simulink model "AvonGasTurbineFAult"  (R2016b)
settings: Solver=ode45  StartTime=0.0  StopTime=3000  FixedStep=1  RelTol=1e-3  EnableMultiTasking=on
InitFcn:
  | warning off
undefined symbols (not defined in the file or in its folder): flagFalut, thresholdbound, xflt
libraries: neural x74, fuzblock x6, simulink x5
(part 3 of 4)

== system AvonGasTurbineFAult/FG_valve/Layer 2/LW{2,1} ==
  "ad{2,1}" : Inport  PortDimensions=10
      mask Display: e = 0.06;c1 = [120 230 180]/255;c2 = ([120 230 180]+0)/(256+128);c3 = ([120 230 180]+128)/(256+128);patch([0 1 1 0],[0 0 1 1],c1);patch([0 1 1 1-e 1-e 0+e],[0 0 1 1-e 0+e 0+e],c2);patch([0 0 1 1-e 0+e 0+e],[0 1 1 1-e 1-e 0+e],c3);plot([0 1 1 0 0],[0 0 1 1 0]);
  "IW{2,1}(1,:)'" : Constant  Value=[-3.0687263870923882;-0.58010050017961035;-1.6732268530537433;1.1111209811250431;-3.7658607876141885;4.9608535154988296;-4.0233887362216931;0.877154954427946;-0.007111666457348894;-2.3567838960567342]
      mask Display: e = 0.06;c1 = [120 150 230]/255;c2 = ([120 150 230]+0)/383;c3 = ([120 150 230]+128)/383;patch([0 1 1 0],[0 0 1 1],c1);patch([0 1 1 1-e 1-e 0+e],[0 0 1 1-e 0+e 0+e],c2);patch([0 0 1 1-e 0+e 0+e],[0 1 1 1-e 1-e 0+e],c3);plot([0 1 1 0 0],[0 0 1 1 0]);disp('weights');
  "IW{2,1}(2,:)'" : Constant  Value=[2.944755261970526;0.25323877938735545;-0.37016123547701313;-0.49590463373628868;-1.4090557527728114;0.65410480645354996;-1.1498049344641088;1.9422996654200746;1.3204846277569529;-1.2106760170631452]
      mask Display: e = 0.06;c1 = [120 150 230]/255;c2 = ([120 150 230]+0)/383;c3 = ([120 150 230]+128)/383;patch([0 1 1 0],[0 0 1 1],c1);patch([0 1 1 1-e 1-e 0+e],[0 0 1 1-e 0+e 0+e],c2);patch([0 0 1 1-e 0+e 0+e],[0 1 1 1-e 1-e 0+e],c3);plot([0 1 1 0 0],[0 0 1 1 0]);disp('weights');
  "IW{2,1}(3,:)'" : Constant  Value=[-0.90291968530259159;1.9861760248636133;-0.86703740713984767;-1.2961573454155009;4.5697519100862136;-0.36889440045356731;2.1467530867666906;-0.28314202170097313;4.7165461441025522;-0.46852595302874794]
      mask Display: e = 0.06;c1 = [120 150 230]/255;c2 = ([120 150 230]+0)/383;c3 = ([120 150 230]+128)/383;patch([0 1 1 0],[0 0 1 1],c1);patch([0 1 1 1-e 1-e 0+e],[0 0 1 1-e 0+e 0+e],c2);patch([0 0 1 1-e 0+e 0+e],[0 1 1 1-e 1-e 0+e],c3);plot([0 1 1 0 0],[0 0 1 1 0]);disp('weights');
  "IW{2,1}(4,:)'" : Constant  Value=[-0.64754745089492727;1.1123312445500233;0.83236734991389205;-1.8490415224064412;1.5705881964870483;-1.0926676182672841;1.6546849856056243;0.32063608320396986;-2.1447230371013397;0.6319277909001263]
      mask Display: e = 0.06;c1 = [120 150 230]/255;c2 = ([120 150 230]+0)/383;c3 = ([120 150 230]+128)/383;patch([0 1 1 0],[0 0 1 1],c1);patch([0 1 1 1-e 1-e 0+e],[0 0 1 1-e 0+e 0+e],c2);patch([0 0 1 1-e 0+e 0+e],[0 1 1 1-e 1-e 0+e],c3);plot([0 1 1 0 0],[0 0 1 1 0]);disp('weights');
  "IW{2,1}(5,:)'" : Constant  Value=[-0.15827585012303017;-3.2384833273086215;3.0202792630042516;1.6954603631555352;-0.30703142185655163;-4.0656025385335557;0.082117475248239757;-2.319580069618365;-2.7902439970303101;2.2531134995583511]
      mask Display: e = 0.06;c1 = [120 150 230]/255;c2 = ([120 150 230]+0)/383;c3 = ([120 150 230]+128)/383;patch([0 1 1 0],[0 0 1 1],c1);patch([0 1 1 1-e 1-e 0+e],[0 0 1 1-e 0+e 0+e],c2);patch([0 0 1 1-e 0+e 0+e],[0 1 1 1-e 1-e 0+e],c3);plot([0 1 1 0 0],[0 0 1 1 0]);disp('weights');
  Mux : Mux  Inputs=5
      mask Display: e = 0.06;c1 = [120 150 230]/255;c2 = ([120 150 230]+0)/383;c3 = ([120 150 230]+128)/383;patch([0 1 1 0],[0 0 1 1],c1);patch([0 1 1 1-e 1-e 0+e],[0 0 1 1-e 0+e 0+e],c2);patch([0 0 1 1-e 0+e 0+e],[0 1 1 1-e 1-e 0+e],c3);plot([0 1 1 0 0],[0 0 1 1 0]);disp('Mux');
  dotprod{1..5} (5 alike) : neural/Weight Functions/dotprod
  "lz{2,1}" : Outport
      mask Display: e = 0.06;c1 = [120 230 180]/255;c2 = ([120 230 180]+0)/(256+128);c3 = ([120 230 180]+128)/(256+128);patch([0 1 1 0],[0 0 1 1],c1);patch([0 1 1 1-e 1-e 0+e],[0 0 1 1-e 0+e 0+e],c2);patch([0 0 1 1-e 0+e 0+e],[0 1 1 1-e 1-e 0+e],c3);plot([0 1 1 0 0],[0 0 1 1 0]);
  wires:
  "IW{2,1}(1,:)'"/1 -> dotprod1/1
  "ad{2,1}"/1 -> dotprod1/2, dotprod2/2, dotprod3/2, dotprod4/2, dotprod5/2
  dotprod1/1 -> Mux/1
  "IW{2,1}(2,:)'"/1 -> dotprod2/1
  dotprod2/1 -> Mux/2
  "IW{2,1}(3,:)'"/1 -> dotprod3/1
  dotprod3/1 -> Mux/3
  "IW{2,1}(4,:)'"/1 -> dotprod4/1
  dotprod4/1 -> Mux/4
  "IW{2,1}(5,:)'"/1 -> dotprod5/1
  dotprod5/1 -> Mux/5
  Mux/1 -> "lz{2,1}"/1

== system AvonGasTurbineFAult/IGV/Layer 1/Delays 1 ==
  "p{1}" : Inport  PortDimensions=4
      mask Display: e = 0.06;c1 = [120 230 180]/255;c2 = ([120 230 180]+0)/(256+128);c3 = ([120 230 180]+128)/(256+128);patch([0 1 1 0],[0 0 1 1],c1);patch([0 1 1 1-e 1-e 0+e],[0 0 1 1-e 0+e 0+e],c2);patch([0 0 1 1-e 0+e 0+e],[0 1 1 1-e 1-e 0+e],c3);plot([0 1 1 0 0],[0 0 1 1 0]);
  mux : Mux  Inputs=1
      mask Display: e = 0.06;c1 = [120 150 230]/255;c2 = ([120 150 230]+0)/383;c3 = ([120 150 230]+128)/383;patch([0 1 1 0],[0 0 1 1],c1);patch([0 1 1 1-e 1-e 0+e],[0 0 1 1-e 0+e 0+e],c2);patch([0 0 1 1-e 0+e 0+e],[0 1 1 1-e 1-e 0+e],c3);plot([0 1 1 0 0],[0 0 1 1 0]);disp('Mux')
  "pd{1,1}" : Outport
      mask Display: e = 0.06;c1 = [120 230 180]/255;c2 = ([120 230 180]+0)/(256+128);c3 = ([120 230 180]+128)/(256+128);patch([0 1 1 0],[0 0 1 1],c1);patch([0 1 1 1-e 1-e 0+e],[0 0 1 1-e 0+e 0+e],c2);patch([0 0 1 1-e 0+e 0+e],[0 1 1 1-e 1-e 0+e],c3);plot([0 1 1 0 0],[0 0 1 1 0]);
  wires:
  "p{1}"/1 -> mux/1
  mux/1 -> "pd{1,1}"/1

== system AvonGasTurbineFAult/IGV/Layer 1/IW{1,1} ==
  "pd{1,1}" : Inport  PortDimensions=4
      mask Display: e = 0.06;c1 = [120 230 180]/255;c2 = ([120 230 180]+0)/(256+128);c3 = ([120 230 180]+128)/(256+128);patch([0 1 1 0],[0 0 1 1],c1);patch([0 1 1 1-e 1-e 0+e],[0 0 1 1-e 0+e 0+e],c2);patch([0 0 1 1-e 0+e 0+e],[0 1 1 1-e 1-e 0+e],c3);plot([0 1 1 0 0],[0 0 1 1 0]);
  "IW{1,1}(1,:)'" : Constant  Value=[2.219594462508871;-7.5031488882774227;-0.16951464085384688;2.2559544534405829]
      mask Display: e = 0.06;c1 = [120 150 230]/255;c2 = ([120 150 230]+0)/383;c3 = ([120 150 230]+128)/383;patch([0 1 1 0],[0 0 1 1],c1);patch([0 1 1 1-e 1-e 0+e],[0 0 1 1-e 0+e 0+e],c2);patch([0 0 1 1-e 0+e 0+e],[0 1 1 1-e 1-e 0+e],c3);plot([0 1 1 0 0],[0 0 1 1 0]);disp('Weights');
  "IW{1,1}(10,:)'" : Constant  Value=[0.72386665044280696;-0.99907541956854495;2.3405431828986853;0.0072098137729970507]
      mask Display: e = 0.06;c1 = [120 150 230]/255;c2 = ([120 150 230]+0)/383;c3 = ([120 150 230]+128)/383;patch([0 1 1 0],[0 0 1 1],c1);patch([0 1 1 1-e 1-e 0+e],[0 0 1 1-e 0+e 0+e],c2);patch([0 0 1 1-e 0+e 0+e],[0 1 1 1-e 1-e 0+e],c3);plot([0 1 1 0 0],[0 0 1 1 0]);disp('Weights');
  "IW{1,1}(2,:)'" : Constant  Value=[0.45828448774301006;0.27635602984492208;-1.8206546653574081;-0.4617645391990064]
      mask Display: e = 0.06;c1 = [120 150 230]/255;c2 = ([120 150 230]+0)/383;c3 = ([120 150 230]+128)/383;patch([0 1 1 0],[0 0 1 1],c1);patch([0 1 1 1-e 1-e 0+e],[0 0 1 1-e 0+e 0+e],c2);patch([0 0 1 1-e 0+e 0+e],[0 1 1 1-e 1-e 0+e],c3);plot([0 1 1 0 0],[0 0 1 1 0]);disp('Weights');
  "IW{1,1}(3,:)'" : Constant  Value=[-1.5611093187654883;-4.7374148655217576;3.4566630566875447;-4.3995088029773095]
      mask Display: e = 0.06;c1 = [120 150 230]/255;c2 = ([120 150 230]+0)/383;c3 = ([120 150 230]+128)/383;patch([0 1 1 0],[0 0 1 1],c1);patch([0 1 1 1-e 1-e 0+e],[0 0 1 1-e 0+e 0+e],c2);patch([0 0 1 1-e 0+e 0+e],[0 1 1 1-e 1-e 0+e],c3);plot([0 1 1 0 0],[0 0 1 1 0]);disp('Weights');
  "IW{1,1}(4,:)'" : Constant  Value=[-0.98908522818625311;5.6378672937480108;-4.3584747443609801;2.7570615027223591]
      mask Display: e = 0.06;c1 = [120 150 230]/255;c2 = ([120 150 230]+0)/383;c3 = ([120 150 230]+128)/383;patch([0 1 1 0],[0 0 1 1],c1);patch([0 1 1 1-e 1-e 0+e],[0 0 1 1-e 0+e 0+e],c2);patch([0 0 1 1-e 0+e 0+e],[0 1 1 1-e 1-e 0+e],c3);plot([0 1 1 0 0],[0 0 1 1 0]);disp('Weights');
  "IW{1,1}(5,:)'" : Constant  Value=[-2.8134324465244105;6.7258882563143096;-2.8661565273937333;1.9718849940549843]
      mask Display: e = 0.06;c1 = [120 150 230]/255;c2 = ([120 150 230]+0)/383;c3 = ([120 150 230]+128)/383;patch([0 1 1 0],[0 0 1 1],c1);patch([0 1 1 1-e 1-e 0+e],[0 0 1 1-e 0+e 0+e],c2);patch([0 0 1 1-e 0+e 0+e],[0 1 1 1-e 1-e 0+e],c3);plot([0 1 1 0 0],[0 0 1 1 0]);disp('Weights');
  "IW{1,1}(6,:)'" : Constant  Value=[0.64902835493212818;-7.9979459495592389;1.9561022488756985;3.6218302495021097]
      mask Display: e = 0.06;c1 = [120 150 230]/255;c2 = ([120 150 230]+0)/383;c3 = ([120 150 230]+128)/383;patch([0 1 1 0],[0 0 1 1],c1);patch([0 1 1 1-e 1-e 0+e],[0 0 1 1-e 0+e 0+e],c2);patch([0 0 1 1-e 0+e 0+e],[0 1 1 1-e 1-e 0+e],c3);plot([0 1 1 0 0],[0 0 1 1 0]);disp('Weights');
  "IW{1,1}(7,:)'" : Constant  Value=[1.1940928536699442;-6.7285372578875018;-3.6315858948149642;9.5498089734393155]
      mask Display: e = 0.06;c1 = [120 150 230]/255;c2 = ([120 150 230]+0)/383;c3 = ([120 150 230]+128)/383;patch([0 1 1 0],[0 0 1 1],c1);patch([0 1 1 1-e 1-e 0+e],[0 0 1 1-e 0+e 0+e],c2);patch([0 0 1 1-e 0+e 0+e],[0 1 1 1-e 1-e 0+e],c3);plot([0 1 1 0 0],[0 0 1 1 0]);disp('Weights');
  "IW{1,1}(8,:)'" : Constant  Value=[1.1941806101782459;1.4326772114463397;3.0251714674031471;-1.0369160912114381]
      mask Display: e = 0.06;c1 = [120 150 230]/255;c2 = ([120 150 230]+0)/383;c3 = ([120 150 230]+128)/383;patch([0 1 1 0],[0 0 1 1],c1);patch([0 1 1 1-e 1-e 0+e],[0 0 1 1-e 0+e 0+e],c2);patch([0 0 1 1-e 0+e 0+e],[0 1 1 1-e 1-e 0+e],c3);plot([0 1 1 0 0],[0 0 1 1 0]);disp('Weights');
  "IW{1,1}(9,:)'" : Constant  Value=[1.4237569579532079;-1.7699786647982259;0.56143834267411519;0.87297028157899992]
      mask Display: e = 0.06;c1 = [120 150 230]/255;c2 = ([120 150 230]+0)/383;c3 = ([120 150 230]+128)/383;patch([0 1 1 0],[0 0 1 1],c1);patch([0 1 1 1-e 1-e 0+e],[0 0 1 1-e 0+e 0+e],c2);patch([0 0 1 1-e 0+e 0+e],[0 1 1 1-e 1-e 0+e],c3);plot([0 1 1 0 0],[0 0 1 1 0]);disp('Weights');
  Mux : Mux  Inputs=10
      mask Display: e = 0.06;c1 = [120 150 230]/255;c2 = ([120 150 230]+0)/383;c3 = ([120 150 230]+128)/383;patch([0 1 1 0],[0 0 1 1],c1);patch([0 1 1 1-e 1-e 0+e],[0 0 1 1-e 0+e 0+e],c2);patch([0 0 1 1-e 0+e 0+e],[0 1 1 1-e 1-e 0+e],c3);plot([0 1 1 0 0],[0 0 1 1 0]);disp('Mux');
  dotprod{1..10} (10 alike) : neural/Weight Functions/dotprod
  "iz{1,1}" : Outport
      mask Display: e = 0.06;c1 = [120 230 180]/255;c2 = ([120 230 180]+0)/(256+128);c3 = ([120 230 180]+128)/(256+128);patch([0 1 1 0],[0 0 1 1],c1);patch([0 1 1 1-e 1-e 0+e],[0 0 1 1-e 0+e 0+e],c2);patch([0 0 1 1-e 0+e 0+e],[0 1 1 1-e 1-e 0+e],c3);plot([0 1 1 0 0],[0 0 1 1 0]);
  wires:
  "IW{1,1}(1,:)'"/1 -> dotprod1/1
  "pd{1,1}"/1 -> dotprod1/2, dotprod2/2, dotprod3/2, dotprod4/2, dotprod5/2, dotprod6/2, dotprod7/2, dotprod8/2, dotprod9/2, dotprod10/2
  dotprod1/1 -> Mux/1
  "IW{1,1}(2,:)'"/1 -> dotprod2/1
  dotprod2/1 -> Mux/2
  "IW{1,1}(3,:)'"/1 -> dotprod3/1
  dotprod3/1 -> Mux/3
  "IW{1,1}(4,:)'"/1 -> dotprod4/1
  dotprod4/1 -> Mux/4
  "IW{1,1}(5,:)'"/1 -> dotprod5/1
  dotprod5/1 -> Mux/5
  "IW{1,1}(6,:)'"/1 -> dotprod6/1
  dotprod6/1 -> Mux/6
  "IW{1,1}(7,:)'"/1 -> dotprod7/1
  dotprod7/1 -> Mux/7
  "IW{1,1}(8,:)'"/1 -> dotprod8/1
  dotprod8/1 -> Mux/8
  "IW{1,1}(9,:)'"/1 -> dotprod9/1
  dotprod9/1 -> Mux/9
  "IW{1,1}(10,:)'"/1 -> dotprod10/1
  dotprod10/1 -> Mux/10
  Mux/1 -> "iz{1,1}"/1

== system AvonGasTurbineFAult/IGV/Layer 2/Delays 1 ==
  "p{2}" : Inport  PortDimensions=10
      mask Display: e = 0.06;c1 = [120 230 180]/255;c2 = ([120 230 180]+0)/(256+128);c3 = ([120 230 180]+128)/(256+128);patch([0 1 1 0],[0 0 1 1],c1);patch([0 1 1 1-e 1-e 0+e],[0 0 1 1-e 0+e 0+e],c2);patch([0 0 1 1-e 0+e 0+e],[0 1 1 1-e 1-e 0+e],c3);plot([0 1 1 0 0],[0 0 1 1 0]);
  mux : Mux  Inputs=1
      mask Display: e = 0.06;c1 = [120 150 230]/255;c2 = ([120 150 230]+0)/383;c3 = ([120 150 230]+128)/383;patch([0 1 1 0],[0 0 1 1],c1);patch([0 1 1 1-e 1-e 0+e],[0 0 1 1-e 0+e 0+e],c2);patch([0 0 1 1-e 0+e 0+e],[0 1 1 1-e 1-e 0+e],c3);plot([0 1 1 0 0],[0 0 1 1 0]);disp('Mux')
  "pd{2,1}" : Outport
      mask Display: e = 0.06;c1 = [120 230 180]/255;c2 = ([120 230 180]+0)/(256+128);c3 = ([120 230 180]+128)/(256+128);patch([0 1 1 0],[0 0 1 1],c1);patch([0 1 1 1-e 1-e 0+e],[0 0 1 1-e 0+e 0+e],c2);patch([0 0 1 1-e 0+e 0+e],[0 1 1 1-e 1-e 0+e],c3);plot([0 1 1 0 0],[0 0 1 1 0]);
  wires:
  "p{2}"/1 -> mux/1
  mux/1 -> "pd{2,1}"/1

== system AvonGasTurbineFAult/IGV/Layer 2/LW{2,1} ==
  "ad{2,1}" : Inport  PortDimensions=10
      mask Display: e = 0.06;c1 = [120 230 180]/255;c2 = ([120 230 180]+0)/(256+128);c3 = ([120 230 180]+128)/(256+128);patch([0 1 1 0],[0 0 1 1],c1);patch([0 1 1 1-e 1-e 0+e],[0 0 1 1-e 0+e 0+e],c2);patch([0 0 1 1-e 0+e 0+e],[0 1 1 1-e 1-e 0+e],c3);plot([0 1 1 0 0],[0 0 1 1 0]);
  "IW{2,1}(1,:)'" : Constant  Value=[3.940586687326959;0.4257788419378471;0.33471481882666088;-5.7498764386280135;-1.4359910880208622;-0.09097117964400607;6.3797145019809625;-0.17650654305267385;-1.4461232423006569;-2.0573826233510557]
      mask Display: e = 0.06;c1 = [120 150 230]/255;c2 = ([120 150 230]+0)/383;c3 = ([120 150 230]+128)/383;patch([0 1 1 0],[0 0 1 1],c1);patch([0 1 1 1-e 1-e 0+e],[0 0 1 1-e 0+e 0+e],c2);patch([0 0 1 1-e 0+e 0+e],[0 1 1 1-e 1-e 0+e],c3);plot([0 1 1 0 0],[0 0 1 1 0]);disp('weights');
  "IW{2,1}(2,:)'" : Constant  Value=[5.8123784210138991;1.1372105140973754;1.4197369429895117;4.8873783244341942;-1.8457344340637254;2.7534724066184726;1.4103636704080826;-0.84251136056997911;-1.2785722332987968;-1.397273122338567]
      mask Display: e = 0.06;c1 = [120 150 230]/255;c2 = ([120 150 230]+0)/383;c3 = ([120 150 230]+128)/383;patch([0 1 1 0],[0 0 1 1],c1);patch([0 1 1 1-e 1-e 0+e],[0 0 1 1-e 0+e 0+e],c2);patch([0 0 1 1-e 0+e 0+e],[0 1 1 1-e 1-e 0+e],c3);plot([0 1 1 0 0],[0 0 1 1 0]);disp('weights');
  "IW{2,1}(3,:)'" : Constant  Value=[-4.8995722885778878;0.41742234616816493;1.313297186852423;-1.7356675930262182;-3.9059928523677643;5.0368249706793682;1.4289064418703283;-1.8354316111465163;-0.79819324027917082;-1.1346564032235094]
      mask Display: e = 0.06;c1 = [120 150 230]/255;c2 = ([120 150 230]+0)/383;c3 = ([120 150 230]+128)/383;patch([0 1 1 0],[0 0 1 1],c1);patch([0 1 1 1-e 1-e 0+e],[0 0 1 1-e 0+e 0+e],c2);patch([0 0 1 1-e 0+e 0+e],[0 1 1 1-e 1-e 0+e],c3);plot([0 1 1 0 0],[0 0 1 1 0]);disp('weights');
  "IW{2,1}(4,:)'" : Constant  Value=[-2.3751293669314428;-0.057413362698049364;-4.2733325424313051;1.6137666963604003;2.9367631124351194;3.051918232975849;-3.9538337666965635;0.49186638767603286;1.4755423377252981;1.6272351967285534]
      mask Display: e = 0.06;c1 = [120 150 230]/255;c2 = ([120 150 230]+0)/383;c3 = ([120 150 230]+128)/383;patch([0 1 1 0],[0 0 1 1],c1);patch([0 1 1 1-e 1-e 0+e],[0 0 1 1-e 0+e 0+e],c2);patch([0 0 1 1-e 0+e 0+e],[0 1 1 1-e 1-e 0+e],c3);plot([0 1 1 0 0],[0 0 1 1 0]);disp('weights');
  "IW{2,1}(5,:)'" : Constant  Value=[-1.5944905166671126;-2.987065005389693;1.7282827088896184;2.5377943244369829;4.2124329183331382;-10.989249055955975;-6.7615447436576739;2.8944778416611809;1.8645049845785233;1.205751399630667]
      mask Display: e = 0.06;c1 = [120 150 230]/255;c2 = ([120 150 230]+0)/383;c3 = ([120 150 230]+128)/383;patch([0 1 1 0],[0 0 1 1],c1);patch([0 1 1 1-e 1-e 0+e],[0 0 1 1-e 0+e 0+e],c2);patch([0 0 1 1-e 0+e 0+e],[0 1 1 1-e 1-e 0+e],c3);plot([0 1 1 0 0],[0 0 1 1 0]);disp('weights');
  Mux : Mux  Inputs=5
      mask Display: e = 0.06;c1 = [120 150 230]/255;c2 = ([120 150 230]+0)/383;c3 = ([120 150 230]+128)/383;patch([0 1 1 0],[0 0 1 1],c1);patch([0 1 1 1-e 1-e 0+e],[0 0 1 1-e 0+e 0+e],c2);patch([0 0 1 1-e 0+e 0+e],[0 1 1 1-e 1-e 0+e],c3);plot([0 1 1 0 0],[0 0 1 1 0]);disp('Mux');
  dotprod{1..5} (5 alike) : neural/Weight Functions/dotprod
  "lz{2,1}" : Outport
      mask Display: e = 0.06;c1 = [120 230 180]/255;c2 = ([120 230 180]+0)/(256+128);c3 = ([120 230 180]+128)/(256+128);patch([0 1 1 0],[0 0 1 1],c1);patch([0 1 1 1-e 1-e 0+e],[0 0 1 1-e 0+e 0+e],c2);patch([0 0 1 1-e 0+e 0+e],[0 1 1 1-e 1-e 0+e],c3);plot([0 1 1 0 0],[0 0 1 1 0]);
  wires:
  "IW{2,1}(1,:)'"/1 -> dotprod1/1
  "ad{2,1}"/1 -> dotprod1/2, dotprod2/2, dotprod3/2, dotprod4/2, dotprod5/2
  dotprod1/1 -> Mux/1
  "IW{2,1}(2,:)'"/1 -> dotprod2/1
  dotprod2/1 -> Mux/2
  "IW{2,1}(3,:)'"/1 -> dotprod3/1
  dotprod3/1 -> Mux/3
  "IW{2,1}(4,:)'"/1 -> dotprod4/1
  dotprod4/1 -> Mux/4
  "IW{2,1}(5,:)'"/1 -> dotprod5/1
  dotprod5/1 -> Mux/5
  Mux/1 -> "lz{2,1}"/1

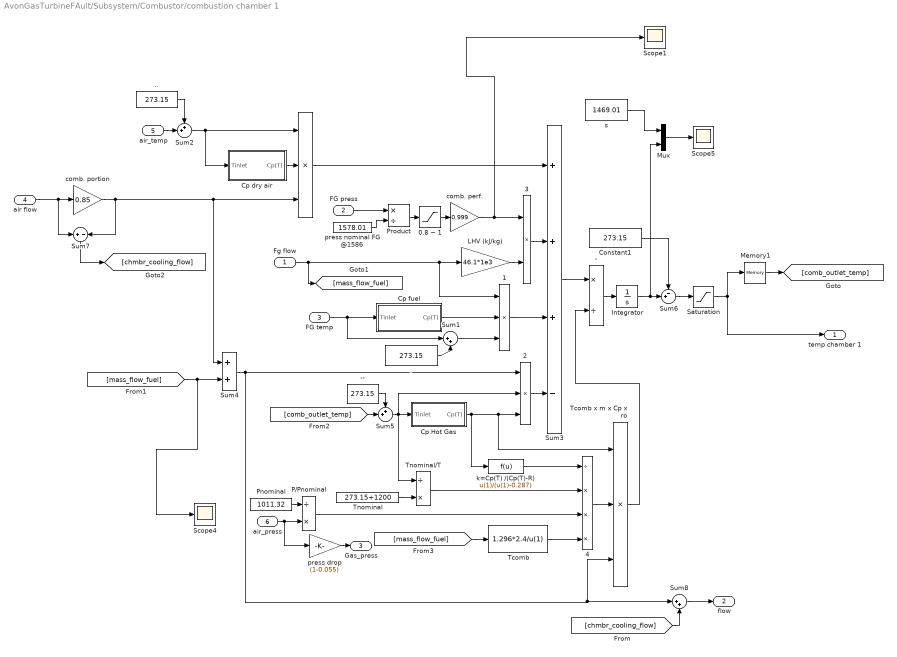
== system AvonGasTurbineFAult/Subsystem/Combustor/combustion chamber 1 ==
  Fg flow : Inport
  FG press : Inport  Port=2
  FG temp : Inport  Port=3
  air flow : Inport  Port=4
  air_temp : Inport  Port=5
  air_press : Inport  Port=6
  "     " : Product  Inputs=3  RndMeth=Zero
  "     1" : Product  Inputs=3  RndMeth=Zero
  "     2" : Product  Inputs=3  RndMeth=Zero
  "     3" : Product  RndMeth=Zero
  "     4" : Product  Inputs=/***  RndMeth=Zero
  " Cp dry air " : Subsystem
  - : Product  Inputs=*/  RndMeth=Zero
  -- : Constant  Value=273.15
  . : Constant  Value=273.15
  .. : Constant  Value=273.15
  0.8 ~ 1 : Saturate  UpperLimit=1  LowerLimit=0.8
  Constant1 : Constant  Value=273.15
  "Cp Hot Gas " : Subsystem
  Cp fuel : Subsystem
  Integrator : Integrator  InitialCondition=780+273.15  LimitOutput=on  UpperSaturationLimit=2000  LowerSaturationLimit=780+273.15
  "LHV (kJ/kg) " : Gain  Gain=46.1*1e3
  Memory1 : Memory  X0=780
  Mux : Mux  Inputs=2
  P/Pnominal : Product  Inputs=/*  RndMeth=Zero
  Pnominal : Constant  Value=1011.32
  Product : Product  Inputs=*/
  Saturation : Saturate  UpperLimit=1400  LowerLimit=350
  Scope1 : Scope
  Scope4 : Scope
  Scope5 : Scope
  Sum1 : Sum  Inputs=|++
  Sum2 : Sum  Inputs=++|
  Sum3 : Sum  Inputs=+++-
  Sum4 : Sum  Inputs=2
  Sum5 : Sum  Inputs=++|
  Sum6 : Sum  Inputs=-+|
  Sum7 : Sum  Inputs=+-
  Sum8 : Sum  Inputs=|++
  Tcomb : Fcn  Expr=1.296*2.4/u(1)  SampleTime=1
  Tcomb x m x Cp x ro : Product  Inputs=3  RndMeth=Zero
  Tnominal : Constant  Value=273.15+1200
  Tnominal/T : Product  Inputs=/*  RndMeth=Zero
  comb. perf. : Gain  Gain=0.999
  comb. portion : Gain  Gain=0.85
  k=Cp(T) /(Cp(T)-R) : Fcn  Expr=u(1)/(u(1)-0.287)
  press drop : Gain  Gain=(1-0.055)  SampleTime=1
  press nominal FG @1586 : Constant  Value=1578.01
  s : Constant  Value=1469.01
  temp chamber 1 : Outport
  flow : Outport  Port=2
  Gas_press : Outport  Port=3
  wires:
  " Cp dry air "/1(Cp(T)) -> "     "/2
  ../1 -> Sum2/1
  Sum2/1 -> " Cp dry air "/1(Tinlet), "     "/1
  FG press/1 -> Product/1
  FG temp/1 -> Sum1/1, Cp fuel/1(Tinlet)
  Sum3/1 -> -/1
  Fg flow/1 -> "     1"/1, "LHV (kJ/kg) "/1, [mass_flow_fuel]
  Sum1/1 -> "     1"/3
  Cp fuel/1(Cp(T)) -> "     1"/2
  "     "/1 -> Sum3/1
  Memory1/1 -> [comb_outlet_temp]
  "     1"/1 -> Sum3/3
  ./1 -> Sum1/2
  "     2"/1 -> Sum3/4
  Tnominal/1 -> Tnominal/T/2
  Sum5/1 -> "     2"/2, "Cp Hot Gas "/1(Tinlet), Tnominal/T/1
  Constant1/1 -> Sum6/1
  Integrator/1 -> Mux/2, Sum6/2
  Sum6/1 -> Saturation/1
  "LHV (kJ/kg) "/1 -> "     3"/2
  Tcomb x m x Cp x ro/1 -> -/2
  Tnominal/T/1 -> "     4"/2
  [mass_flow_fuel] -> Scope4/1, Sum4/2
  "Cp Hot Gas "/1(Cp(T)) -> k=Cp(T) /(Cp(T)-R)/1, "     2"/3, Tcomb x m x Cp x ro/1
  --/1 -> Sum5/1
  Pnominal/1 -> P/Pnominal/1
  air_press/1 -> press drop/1, P/Pnominal/2
  "     4"/1 -> Tcomb x m x Cp x ro/2
  k=Cp(T) /(Cp(T)-R)/1 -> "     4"/1
  [comb_outlet_temp] -> Sum5/2
  P/Pnominal/1 -> "     4"/3
  air_temp/1 -> Sum2/2
  -/1 -> Integrator/1
  Saturation/1 -> temp chamber 1/1, Memory1/1
  s/1 -> Mux/1
  Sum4/1 -> "     2"/1, Sum8/1, Tcomb x m x Cp x ro/3
  Mux/1 -> Scope5/1
  press drop/1 -> Gas_press/1
  press nominal FG @1586/1 -> Product/2
  Product/1 -> 0.8 ~ 1/1
  0.8 ~ 1/1 -> comb. perf./1
  comb. perf./1 -> "     3"/1, Scope1/1
  "     3"/1 -> Sum3/2
  [mass_flow_fuel] -> Tcomb/1
  Tcomb/1 -> "     4"/4
  air flow/1 -> Sum7/1, comb. portion/1
  comb. portion/1 -> Sum7/2, "     "/3, Sum4/1
  Sum8/1 -> flow/1
  [chmbr_cooling_flow] -> Sum8/2
  Sum7/1 -> [chmbr_cooling_flow]

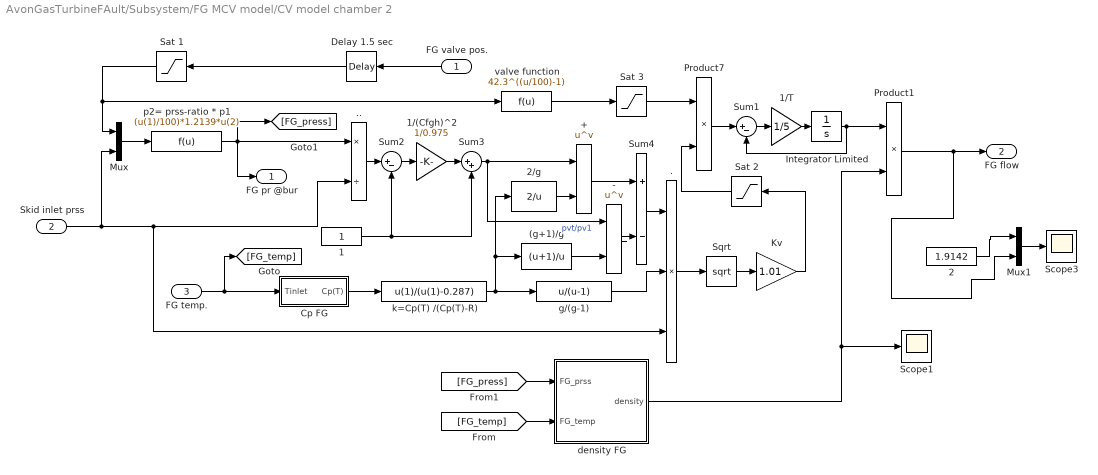
== system AvonGasTurbineFAult/Subsystem/FG MCV model/CV model chamber 2 ==
  FG valve pos. : Inport
  Skid inlet prss : Inport  Port=2
  FG temp. : Inport  Port=3
  "  (g+1)/g" : Fcn  Expr=(u+1)/u
  "  Sqrt  " : Sqrt  SaturateOnIntegerOverflow=on
  " k=Cp(T) /(Cp(T)-R) " : Fcn  Expr=u(1)/(u(1)-0.287)
  + : Math  Operator=pow  SaturateOnIntegerOverflow=on
  - : Math  Operator=pow  SaturateOnIntegerOverflow=on
  . : Product  Inputs=3  RndMeth=Zero
  .. : Product  Inputs=*/  RndMeth=Zero
  1 : Constant
  1/(Cfgh)^2 : Gain  Gain=1/0.975
  1/T : Gain  Gain=1/5
  2 : Constant  Value=1.9142
  2/g : Fcn  Expr=2/u
  Cp FG : Subsystem
  Delay 1.5 sec : TransportDelay  DelayTime=1.5  InitialOutput=30
  Integrator Limited : Integrator  InitialCondition=1.9  LimitOutput=on  UpperSaturationLimit=5  LowerSaturationLimit=0.01
  Kv : Gain  Gain=1.01
  Mux : Mux  Inputs=2
  Mux1 : Mux  Inputs=2
  Product1 : Product  RndMeth=Zero
  Product7 : Product  RndMeth=Zero
  Sat 1 : Saturate  UpperLimit=100  LowerLimit=0.01
  Sat 2 : Saturate  UpperLimit=300  LowerLimit=0.001
  Sat 3 : Saturate  UpperLimit=1  LowerLimit=0.01
  Scope1 : Scope
  Scope3 : Scope
  Sum1 : Sum  Inputs=|+-
  Sum2 : Sum  Inputs=|+-
  Sum3 : Sum  Inputs=|++
  Sum4 : Sum  Inputs=+-
  density FG : Subsystem
  g/(g-1) : Fcn  Expr=u/(u-1)
  p2= prss-ratio * p1 : Fcn  Expr=(u(1)/100)*1.2139*u(2)  SampleTime=1
  valve function : Fcn  Expr=42.3^((u/100)-1)  SampleTime=1
  FG pr @bur : Outport
  FG flow : Outport  Port=2
  wires:
  Sat 2/1 -> Product7/2
  Sum3/1 -> +/1, -/1  "pvt/pv1"
  Sum4/1 -> ./1
  "  Sqrt  "/1 -> Kv/1
  ../1 -> Sum2/1
  Skid inlet prss/1 -> ../2, ./3, Mux/2
  2/g/1 -> +/2
  1/(Cfgh)^2/1 -> Sum3/1
  Sum2/1 -> 1/(Cfgh)^2/1
  FG temp./1 -> [FG_temp], Cp FG/1(Tinlet)
  "  (g+1)/g"/1 -> -/2
  -/1 -> Sum4/2
  " k=Cp(T) /(Cp(T)-R) "/1 -> g/(g-1)/1, "  (g+1)/g"/1, 2/g/1
  g/(g-1)/1 -> ./2
  p2= prss-ratio * p1/1 -> [FG_press], ../1, FG pr @bur/1
  +/1 -> Sum4/1
  1/1 -> Sum3/2, Sum2/2
  Cp FG/1(Cp(T)) -> " k=Cp(T) /(Cp(T)-R) "/1
  Mux/1 -> p2= prss-ratio * p1/1
  valve function/1 -> Sat 3/1
  FG valve pos./1 -> Delay 1.5 sec/1
  Delay 1.5 sec/1 -> Sat 1/1
  Sat 1/1 -> Mux/1, valve function/1
  Sat 3/1 -> Product7/1
  Kv/1 -> Sat 2/1
  Sum1/1 -> 1/T/1
  1/T/1 -> Integrator Limited/1
  Integrator Limited/1 -> Product1/1, Sum1/2
  ./1 -> "  Sqrt  "/1
  Product7/1 -> Sum1/1
  [FG_temp] -> density FG/2(FG_temp)
  [FG_press] -> density FG/1(FG_prss)
  density FG/1(density) -> Scope1/1, Product1/2
  Mux1/1 -> Scope3/1
  Product1/1 -> Mux1/2, FG flow/1
  2/1 -> Mux1/1

== system AvonGasTurbineFAult/Subsystem/FG MCV model/Subsystem1 ==
  gas prss : Inport
  FG temp. : Inport  Port=2
  FG flow : Inport  Port=3
  " 2 " : Constant  Value=2
  . : Product  Inputs=3  RndMeth=Zero
  2 : Constant  Value=2
  Kf : Gain  Gain=16.8993
  Math Function5 : Math  Operator=pow  SaturateOnIntegerOverflow=on
  Memory : Memory
  Sqrt : Sqrt  SaturateOnIntegerOverflow=on
  Sqrt1 : Sqrt  SaturateOnIntegerOverflow=on
  Sqrt2 : Sqrt  SaturateOnIntegerOverflow=on
  Sum1 : Sum  Inputs=-+|
  Sum5 : Sum  Inputs=|++
  Sum9 : Sum  Inputs=|+-
  Z : Subsystem
  c4 : Constant  Value=273.15
  n flow exp. : Constant  Value=0.4835
  pressure drop 5 kPa : Constant  Value=5
  pw : Math  Operator=pow  SaturateOnIntegerOverflow=on
  pw1 : Math  Operator=pow  SaturateOnIntegerOverflow=on
  " FG skid inlet prss" : Outport
  skid temp : Outport  Port=2
  wires:
  pressure drop 5 kPa/1 -> Sum1/1
  Sum1/1 -> pw1/1
  Sqrt1/1 -> ./3
  Memory/1 -> Z/2(P)
  Sqrt/1 -> ./2
  Sum5/1 -> Z/1(T), Sqrt/1
  c4/1 -> Sum5/2
  Z/1(Z) -> Sqrt1/1
  Sqrt2/1 -> Memory/1, " FG skid inlet prss"/1
  Math Function5/1 -> ./1
  FG flow/1 -> Math Function5/1
  n flow exp./1 -> Math Function5/2
  pw/1 -> Sum9/2
  2/1 -> pw/2
  Sum9/1 -> Sqrt2/1
  pw1/1 -> Sum9/1
  Kf/1 -> pw/1
  ./1 -> Kf/1
  FG temp./1 -> Sum5/1, skid temp/1
  " 2 "/1 -> pw1/2
  gas prss/1 -> Sum1/2

== system AvonGasTurbineFAult/Subsystem/Subsystem1/Cp @ trb. input ==
  Tinlet : Inport
  Cp : Fcn  Expr=(3.355+5.75*1e-4*u(1)-1600*u(1)^(-2))*0.28714  SampleTime=1
  Cp(T) : Outport
  wires:
  Cp/1 -> Cp(T)/1
  Tinlet/1 -> Cp/1

== system AvonGasTurbineFAult/Subsystem/Subsystem1/Cp @ trb. output ==
  Tinlet : Inport
  Cp : Fcn  Expr=(3.355+5.75*1e-4*u(1)-1600*u(1)^(-2))*0.28714  SampleTime=1
  Cp(T) : Outport
  wires:
  Tinlet/1 -> Cp/1
  Cp/1 -> Cp(T)/1

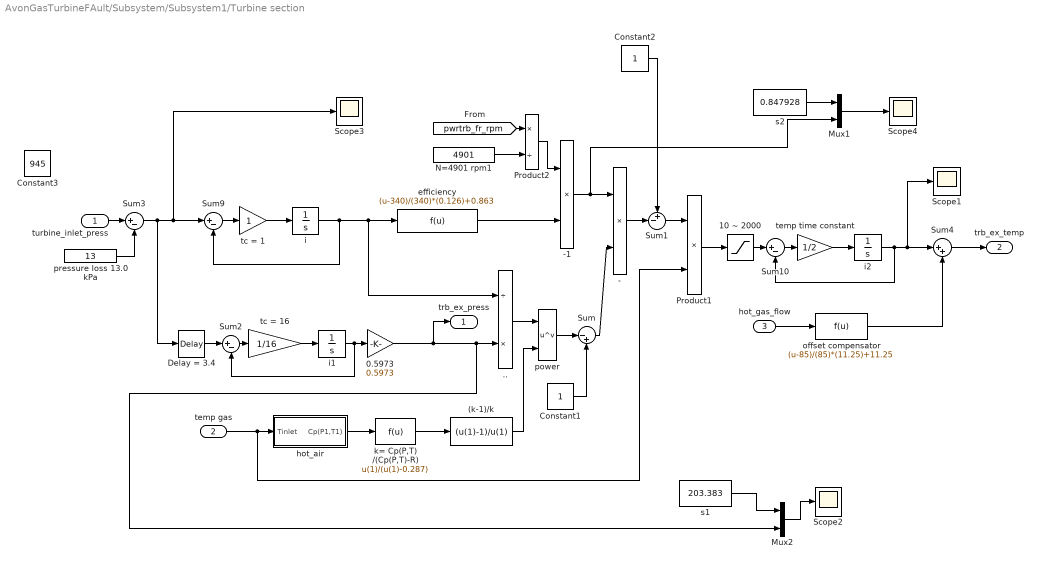
== system AvonGasTurbineFAult/Subsystem/Subsystem1/Turbine section ==
  turbine_inlet_press : Inport
  temp gas : Inport  Port=2
  hot_gas_flow : Inport  Port=3
  (k-1)/k : Fcn  Expr=(u(1)-1)/u(1)
  - : Product  RndMeth=Zero
  -1 : Product  RndMeth=Zero
  .. : Product  Inputs=/*  RndMeth=Zero
  0.5973 : Gain  Gain=0.5973
  10 ~ 2000 : Saturate  UpperLimit=2000  LowerLimit=10
  Constant1 : Constant
  Constant2 : Constant
  Constant3 : Constant  Value=945
  Delay = 3.4 : TransportDelay  DelayTime=3.4  InitialOutput=230.380
  Mux1 : Mux  Inputs=2
  Mux2 : Mux  Inputs=2
  N=4901 rpm1 : Constant  Value=4901
  Product1 : Product  RndMeth=Zero
  Product2 : Product  Inputs=*/  RndMeth=Zero
  Scope{1..4} (4 alike) : Scope
  Sum : Sum  Inputs=|-+
  Sum1 : Sum  Inputs=+-|
  Sum{2..3,9..10} (4 alike) : Sum  Inputs=|+-
  Sum4 : Sum  Inputs=|++
  efficiency : Fcn  Expr=(u-340)/(340)*(0.126)+0.863
  hot_air : Subsystem
  i : Integrator  InitialCondition=340  LimitOutput=on  UpperSaturationLimit=1000  LowerSaturationLimit=1
  i1 : Integrator  InitialCondition=203  LimitOutput=on  UpperSaturationLimit=500  LowerSaturationLimit=1
  i2 : Integrator  InitialCondition=1082  LimitOutput=on  UpperSaturationLimit=2000  LowerSaturationLimit=400
  k= Cp(P,T) /(Cp(P,T)-R) : Fcn  Expr=u(1)/(u(1)-0.287)
  offset compensator : Fcn  Expr=(u-85)/(85)*(11.25)+11.25  SampleTime=1
  power : Math  Operator=pow  SaturateOnIntegerOverflow=on
  pressure loss 13.0 kPa : Constant  Value=13
  s1 : Constant  Value=203.383
  s2 : Constant  Value=0.847928
  tc = 1 : Gain
  tc = 16 : Gain  Gain=1/16
  temp time constant : Gain  Gain=1/2
  trb_ex_press : Outport
  trb_ex_temp : Outport  Port=2
  wires:
  ../1 -> power/1
  turbine_inlet_press/1 -> Sum3/1
  tc = 16/1 -> i1/1
  Sum2/1 -> tc = 16/1
  i1/1 -> 0.5973/1, Sum2/2
  s2/1 -> Mux1/1
  Mux1/1 -> Scope4/1
  i2/1 -> Sum10/2, Sum4/1, Scope1/1
  10 ~ 2000/1 -> Sum10/1
  temp gas/1 -> hot_air/1(Tinlet), Product1/2
  Sum1/1 -> Product1/1
  Constant2/1 -> Sum1/1
  pressure loss 13.0 kPa/1 -> Sum3/2
  Product1/1 -> 10 ~ 2000/1
  temp time constant/1 -> i2/1
  Sum10/1 -> temp time constant/1
  tc = 1/1 -> i/1
  Sum9/1 -> tc = 1/1
  Sum/1 -> -/2
  (k-1)/k/1 -> power/2
  hot_air/1(Cp(P1,T1)) -> k= Cp(P,T) /(Cp(P,T)-R)/1
  k= Cp(P,T) /(Cp(P,T)-R)/1 -> (k-1)/k/1
  Sum3/1 -> Scope3/1, Sum9/1, Delay = 3.4/1
  -/1 -> Sum1/2
  Constant1/1 -> Sum/2
  power/1 -> Sum/1
  i/1 -> efficiency/1, ../1, Sum9/2
  s1/1 -> Mux2/1
  Mux2/1 -> Scope2/1
  offset compensator/1 -> Sum4/2
  hot_gas_flow/1 -> offset compensator/1
  Sum4/1 -> trb_ex_temp/1
  0.5973/1 -> trb_ex_press/1, Mux2/2, ../2
  N=4901 rpm1/1 -> Product2/2
  [pwrtrb_fr_rpm] -> Product2/1
  Product2/1 -> -1/1
  -1/1 -> Mux1/2, -/1
  Delay = 3.4/1 -> Sum2/1
  efficiency/1 -> -1/2

== system AvonGasTurbineFAult/Subsystem/Subsystem1/rotor dynamic ==
  gen_turb : Inport
  consm_comp : Inport  Port=2
  ...1 : Product  Inputs=*/
  ...2 : Product  Inputs=/*
  ...3 : Product
  F1 : Constant  Value=87
  Gain1 : Gain  Gain=0.5
  Gain2 : Gain  Gain=30/pi
  Gain4 : Gain  Gain=pi/30
  Integrator1 : Integrator  InitialCondition=pi/30*4901  LimitOutput=on  UpperSaturationLimit=4900*1.20  LowerSaturationLimit=0.01
  J_rotor1 : Gain  Gain=1/51
  Loss : Gain  Gain=0.01
  Math Function : Math  Operator=square  SaturateOnIntegerOverflow=on
  Memory Omega2 : Memory  X0=pi/30*4901
  Mux4 : Mux  Inputs=2
  Product1 : Product  Inputs=*/
  Scope1 : Scope
  Scope8 : Scope
  Scope9 : Scope
  Sum3 : Sum  Inputs=++|
  Sum7 : Sum  Inputs=|++
  Sum8 : Sum  Inputs=|+-
  Sum9 : Sum  Inputs=|+-
  freq_rotor2 : Constant
  freq_rotor3 : Constant  Value=4901
  power1 : Constant  Value=4901
  rotor_speed : Outport
  wires:
  Sum9/1 -> ...1/1
  Memory Omega2/1 -> Sum7/2
  Gain4/1 -> ...2/1, Sum7/1
  Sum7/1 -> ...2/2, ...1/2
  ...3/1 -> J_rotor1/1
  ...1/1 -> ...3/2
  J_rotor1/1 -> Integrator1/1
  Loss/1 -> Sum9/2
  consm_comp/1 -> Sum8/2
  Sum8/1 -> Scope8/1, Sum9/1
  ...2/1 -> Math Function/1
  Gain1/1 -> ...3/1, Scope1/1
  Math Function/1 -> Loss/1
  Integrator1/1 -> Memory Omega2/1, rotor_speed/1, Gain2/1
  power1/1 -> Mux4/2
  Mux4/1 -> Scope9/1
  Gain2/1 -> Mux4/1
  gen_turb/1 -> Sum8/1
  freq_rotor3/1 -> Gain4/1
  F1/1 -> Product1/2
  [gg_flow] -> Product1/1
  Product1/1 -> Sum3/1
  freq_rotor2/1 -> Sum3/2
  Sum3/1 -> Gain1/1

== system AvonGasTurbineFAult/Subsystem/Subsystem2/Cp @ trb. input ==
  Tinlet : Inport
  Cp : Fcn  Expr=(3.355+5.75*1e-4*u(1)-1600*u(1)^(-2))*0.28714  SampleTime=1
  Cp(T) : Outport
  wires:
  Tinlet/1 -> Cp/1
  Cp/1 -> Cp(T)/1

== system AvonGasTurbineFAult/Subsystem/Subsystem2/Cp @ trb. output ==
  Tinlet : Inport
  Cp : Fcn  Expr=(3.355+5.75*1e-4*u(1)-1600*u(1)^(-2))*0.28714  SampleTime=1
  Cp(T) : Outport
  wires:
  Cp/1 -> Cp(T)/1
  Tinlet/1 -> Cp/1

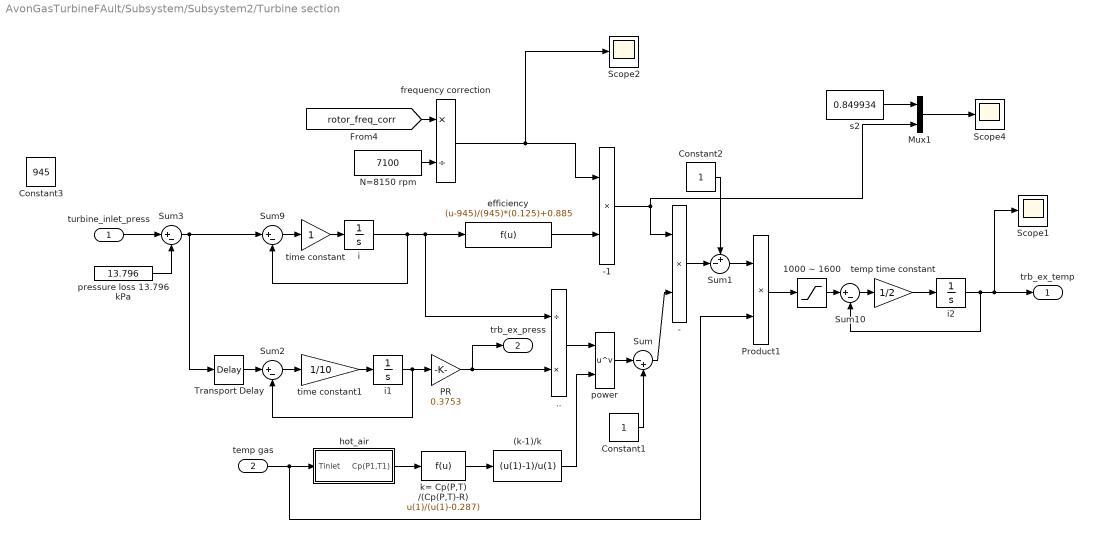
== system AvonGasTurbineFAult/Subsystem/Subsystem2/Turbine section ==
  turbine_inlet_press : Inport
  temp gas : Inport  Port=2
  (k-1)/k : Fcn  Expr=(u(1)-1)/u(1)
  - : Product  RndMeth=Zero
  -1 : Product  RndMeth=Zero
  .. : Product  Inputs=/*  RndMeth=Zero
  1000 ~ 1600 : Saturate  UpperLimit=2000  LowerLimit=400
  Constant1 : Constant
  Constant2 : Constant
  Constant3 : Constant  Value=945
  Mux1 : Mux  Inputs=2
  N=8150 rpm : Constant  Value=7100
  PR : Gain  Gain=0.3753
  Product1 : Product  RndMeth=Zero
  Scope1 : Scope
  Scope2 : Scope
  Scope4 : Scope
  Sum : Sum  Inputs=|-+
  Sum1 : Sum  Inputs=+-|
  Sum{2..3,9..10} (4 alike) : Sum  Inputs=|+-
  Transport Delay : TransportDelay  DelayTime=1.6  InitialOutput=941.9108
  efficiency : Fcn  Expr=(u-945)/(945)*(0.125)+0.885
  frequency correction : Product  Inputs=*/  RndMeth=Zero
  hot_air : Subsystem
  i : Integrator  InitialCondition=507  LimitOutput=on  UpperSaturationLimit=1100  LowerSaturationLimit=10
  i1 : Integrator  InitialCondition=507  LimitOutput=on  UpperSaturationLimit=1100  LowerSaturationLimit=500
  i2 : Integrator  InitialCondition=450+273.15  LimitOutput=on  UpperSaturationLimit=2000  LowerSaturationLimit=400
  k= Cp(P,T) /(Cp(P,T)-R) : Fcn  Expr=u(1)/(u(1)-0.287)
  power : Math  Operator=pow  SaturateOnIntegerOverflow=on
  pressure loss 13.796 kPa : Constant  Value=13.796
  s2 : Constant  Value=0.849934
  temp time constant : Gain  Gain=1/2
  time constant : Gain
  time constant1 : Gain  Gain=1/10
  trb_ex_temp : Outport
  trb_ex_press : Outport  Port=2
  wires:
  i/1 -> Sum9/2, efficiency/1, ../1
  power/1 -> Sum/1
  Constant1/1 -> Sum/2
  -/1 -> Sum1/2
  Sum3/1 -> Sum9/1, Transport Delay/1
  k= Cp(P,T) /(Cp(P,T)-R)/1 -> (k-1)/k/1
  hot_air/1(Cp(P1,T1)) -> k= Cp(P,T) /(Cp(P,T)-R)/1
  (k-1)/k/1 -> power/2
  Sum/1 -> -/2
  Sum9/1 -> time constant/1
  time constant/1 -> i/1
  Sum10/1 -> temp time constant/1
  temp time constant/1 -> i2/1
  Product1/1 -> 1000 ~ 1600/1
  pressure loss 13.796 kPa/1 -> Sum3/2
  Constant2/1 -> Sum1/1
  Sum1/1 -> Product1/1
  temp gas/1 -> hot_air/1(Tinlet), Product1/2
  1000 ~ 1600/1 -> Sum10/1
  i2/1 -> Scope1/1, trb_ex_temp/1, Sum10/2
  Mux1/1 -> Scope4/1
  s2/1 -> Mux1/1
  -1/1 -> -/1, Mux1/2
  i1/1 -> Sum2/2, PR/1
  Sum2/1 -> time constant1/1
  time constant1/1 -> i1/1
  turbine_inlet_press/1 -> Sum3/1
  PR/1 -> trb_ex_press/1, ../2
  ../1 -> power/1
  Transport Delay/1 -> Sum2/1
  N=8150 rpm/1 -> frequency correction/2
  [rotor_freq_corr] -> frequency correction/1
  efficiency/1 -> -1/2
  frequency correction/1 -> Scope2/1, -1/1

== system AvonGasTurbineFAult/Subsystem/Subsystem2/cooling 1 ==
  cooling_air_temp : Inport
  cooling_air_flow : Inport  Port=2
  hot_gas_flow : Inport  Port=3
  hot_gas_temp : Inport  Port=4
  "     1" : Product  RndMeth=Zero
  "     2" : Product  Inputs=3  RndMeth=Zero
  "     4" : Product  Inputs=3  RndMeth=Zero
  . : Product  Inputs=*/  RndMeth=Zero
  Cp Temp : Subsystem
  Cp Temp air : Subsystem
  Cp Temp hot gas : Subsystem
  Integrator : Integrator  InitialCondition=765+273.15+12  LimitOutput=on  UpperSaturationLimit=1250+273.15  LowerSaturationLimit=600+273.15
  Memory : Memory  X0=750+273.15
  Scope1 : Scope
  Sum1 : Sum  Inputs=2
  Sum2 : Sum  Inputs=2
  Sum6 : Sum  Inputs=|+-
  time constant : Gain  Gain=1/3.6
  temp gas : Outport
  gas_flow : Outport  Port=2
  wires:
  hot_gas_temp/1 -> Cp Temp hot gas/1(Tinlet), "     4"/2
  hot_gas_flow/1 -> Sum1/1, "     4"/1
  Cp Temp hot gas/1(Cp(T)) -> "     4"/3
  cooling_air_temp/1 -> Cp Temp air/1(Tinlet), "     2"/2
  cooling_air_flow/1 -> Sum1/2, "     2"/1
  Cp Temp air/1(Cp(T)) -> "     2"/3
  "     2"/1 -> Sum2/1
  "     4"/1 -> Sum2/2
  Sum2/1 -> ./1
  Cp Temp/1(Cp(T)) -> "     1"/2
  Memory/1 -> Cp Temp/1(Tinlet)
  "     1"/1 -> ./2
  ./1 -> Sum6/1
  time constant/1 -> Integrator/1
  Sum6/1 -> time constant/1
  Integrator/1 -> temp gas/1, Scope1/1, Sum6/2, Memory/1
  Sum1/1 -> "     1"/1, gas_flow/1

== system AvonGasTurbineFAult/Subsystem/Subsystem2/cooling 2 ==
  cooling_air_temp : Inport
  cooling_air_flow : Inport  Port=2
  hot_gas_flow : Inport  Port=3
  hot_gas_temp : Inport  Port=4
  "     1" : Product  RndMeth=Zero
  "     2" : Product  Inputs=3  RndMeth=Zero
  "     4" : Product  Inputs=3  RndMeth=Zero
  . : Product  Inputs=*/  RndMeth=Zero
  Constant : Constant  Value=-600
  Cp Temp : Subsystem
  Cp Temp air : Subsystem
  Cp Temp hot gas : Subsystem
  Integrator : Integrator  InitialCondition=1204.4  LimitOutput=on  UpperSaturationLimit=2000  LowerSaturationLimit=100
  Memory : Memory  X0=500+273.15
  Scope1 : Scope
  Scope4 : Scope
  Sum1 : Sum  Inputs=2
  Sum2 : Sum  Inputs=2
  Sum3 : Sum  Inputs=++|
  Sum6 : Sum  Inputs=|+-
  Sum7 : Sum  Inputs=|++
  offset compensator1 : Fcn  Expr=(u-87)/(87)*(14.48)-14.45
  time constant : Gain  Gain=1/5
  gas_flow : Outport
  temp turb : Outport  Port=2
  temp exh turb : Outport  Port=3
  wires:
  Sum6/1 -> time constant/1
  time constant/1 -> Integrator/1
  ./1 -> Sum6/1
  "     1"/1 -> ./2
  Memory/1 -> Cp Temp/1(Tinlet)
  Cp Temp/1(Cp(T)) -> "     1"/2
  Sum1/1 -> Scope4/1, gas_flow/1, "     1"/1, offset compensator1/1
  Sum2/1 -> ./1
  "     4"/1 -> Sum2/2
  "     2"/1 -> Sum2/1
  Cp Temp air/1(Cp(T)) -> "     2"/3
  cooling_air_flow/1 -> "     2"/1, Sum1/2
  cooling_air_temp/1 -> "     2"/2, Cp Temp air/1(Tinlet)
  Cp Temp hot gas/1(Cp(T)) -> "     4"/3
  hot_gas_flow/1 -> "     4"/1, Sum1/1
  hot_gas_temp/1 -> "     4"/2, Cp Temp hot gas/1(Tinlet), Sum3/1
  Integrator/1 -> Sum7/1, Scope1/1, Sum6/2, Memory/1
  Sum3/1 -> temp turb/1
  offset compensator1/1 -> Sum3/2
  Sum7/1 -> temp exh turb/1

== system AvonGasTurbineFAult/Subsystem/Subsystem2/rotor dynamic  ==
  gen_turb : Inport
  consm_comp : Inport  Port=2
  ...1 : Product  Inputs=*/
  ...2 : Product  Inputs=/*
  ...3 : Product
  F1 : Constant  Value=1.9141
  Gain1 : Gain  Gain=0.5
  Gain2 : Gain  Gain=30/pi
  Gain4 : Gain  Gain=pi/30
  Integrator1 : Integrator  InitialCondition=pi/30*7250  LimitOutput=on  UpperSaturationLimit=1200  LowerSaturationLimit=0.01
  J_rotor1 : Gain  Gain=1/60
  Loss : Gain  Gain=0.001
  Math Function : Math  Operator=square  SaturateOnIntegerOverflow=on
  Memory Omega2 : Memory  X0=pi/30*7250
  Mux4 : Mux  Inputs=2
  Product2 : Product  Inputs=*/
  Scope1 : Scope
  Scope8 : Scope
  Scope9 : Scope
  Sum1 : Sum  Inputs=++|
  Sum7 : Sum  Inputs=|++
  Sum8 : Sum  Inputs=|+-
  Sum9 : Sum  Inputs=|+-
  freq_rotor2 : Constant
  freq_rotor3 : Constant  Value=7250
  power1 : Constant  Value=7250
  rotor_speed : Outport
  wires:
  F1/1 -> Product2/2
  Memory Omega2/1 -> Sum7/2
  Gain4/1 -> ...2/1, Sum7/1
  Sum7/1 -> ...2/2, ...1/2
  [FG_flow] -> Product2/1
  freq_rotor3/1 -> Gain4/1
  J_rotor1/1 -> Integrator1/1
  Loss/1 -> Sum9/2
  consm_comp/1 -> Sum8/2
  Sum8/1 -> Scope8/1, Sum9/1
  ...2/1 -> Math Function/1
  Math Function/1 -> Loss/1
  Integrator1/1 -> Gain2/1, Memory Omega2/1, rotor_speed/1
  power1/1 -> Mux4/2
  Mux4/1 -> Scope9/1
  Gain2/1 -> Mux4/1
  gen_turb/1 -> Sum8/1
  Sum9/1 -> ...1/1
  ...1/1 -> ...3/2
  ...3/1 -> J_rotor1/1
  Product2/1 -> Sum1/1
  Gain1/1 -> Scope1/1, ...3/1
  freq_rotor2/1 -> Sum1/2
  Sum1/1 -> Gain1/1

== system AvonGasTurbineFAult/Subsystem/comp_temp/Cp @Cop Outlet ==
  Tinlet : Inport
  Cp : Fcn  Expr=(3.355+5.75*1e-4*u(1)-1600*u(1)^(-2))*0.28714  SampleTime=1
  oC-----> K : Fcn  Expr=(u(1)+273.15)  SampleTime=1
  Cp(T) : Outport
  wires:
  oC-----> K/1 -> Cp/1
  Cp/1 -> Cp(T)/1
  Tinlet/1 -> oC-----> K/1

== system AvonGasTurbineFAult/Subsystem/comp_temp/Cp_com_in ==
  humidity ratio : Inport
  pressuer : Inport  Port=2
  temp. : Inport  Port=3
  .1 : Product  RndMeth=Zero
  .2 : Product  RndMeth=Zero
  Cp dry air : Subsystem
  Cp steam : Subsystem
  R dry air : Constant  Value=0.287
  R steam : Constant  Value=0.4615
  Specific humidity : Subsystem
  Sum1 : Sum  Inputs=++|
  Sum4 : Sum  Inputs=|++
  Cp : Outport
  Rwet : Outport  Port=2
  wires:
  .1/1 -> Sum4/1
  Specific humidity/1(y) -> .2/2, .1/1
  Cp steam/1(Cp(T)) -> .1/2
  Cp dry air/1(Cp(T)) -> Sum4/2
  humidity ratio/1 -> Specific humidity/1(humidity)
  pressuer/1 -> Specific humidity/2(Press_kPa)
  Sum4/1 -> Cp/1
  temp./1 -> Specific humidity/3(temp), Cp steam/1(Tinlet), Cp dry air/1(Tinlet)
  R steam/1 -> .2/1
  .2/1 -> Sum1/2
  Sum1/1 -> Rwet/1
  R dry air/1 -> Sum1/1

== system AvonGasTurbineFAult/comp performance/Layer 1/Delays 1 ==
  "p{1}" : Inport  PortDimensions=6
      mask Display: e = 0.06;c1 = [120 230 180]/255;c2 = ([120 230 180]+0)/(256+128);c3 = ([120 230 180]+128)/(256+128);patch([0 1 1 0],[0 0 1 1],c1);patch([0 1 1 1-e 1-e 0+e],[0 0 1 1-e 0+e 0+e],c2);patch([0 0 1 1-e 0+e 0+e],[0 1 1 1-e 1-e 0+e],c3);plot([0 1 1 0 0],[0 0 1 1 0]);
  mux : Mux  Inputs=1
      mask Display: e = 0.06;c1 = [120 150 230]/255;c2 = ([120 150 230]+0)/383;c3 = ([120 150 230]+128)/383;patch([0 1 1 0],[0 0 1 1],c1);patch([0 1 1 1-e 1-e 0+e],[0 0 1 1-e 0+e 0+e],c2);patch([0 0 1 1-e 0+e 0+e],[0 1 1 1-e 1-e 0+e],c3);plot([0 1 1 0 0],[0 0 1 1 0]);disp('Mux')
  "pd{1,1}" : Outport
      mask Display: e = 0.06;c1 = [120 230 180]/255;c2 = ([120 230 180]+0)/(256+128);c3 = ([120 230 180]+128)/(256+128);patch([0 1 1 0],[0 0 1 1],c1);patch([0 1 1 1-e 1-e 0+e],[0 0 1 1-e 0+e 0+e],c2);patch([0 0 1 1-e 0+e 0+e],[0 1 1 1-e 1-e 0+e],c3);plot([0 1 1 0 0],[0 0 1 1 0]);
  wires:
  "p{1}"/1 -> mux/1
  mux/1 -> "pd{1,1}"/1

== system AvonGasTurbineFAult/comp performance/Layer 1/IW{1,1} ==
  "pd{1,1}" : Inport  PortDimensions=6
      mask Display: e = 0.06;c1 = [120 230 180]/255;c2 = ([120 230 180]+0)/(256+128);c3 = ([120 230 180]+128)/(256+128);patch([0 1 1 0],[0 0 1 1],c1);patch([0 1 1 1-e 1-e 0+e],[0 0 1 1-e 0+e 0+e],c2);patch([0 0 1 1-e 0+e 0+e],[0 1 1 1-e 1-e 0+e],c3);plot([0 1 1 0 0],[0 0 1 1 0]);
  "IW{1,1}(1,:)'" : Constant  Value=[1.5711511404281731;-2.228813602852155;-3.194874552727383;-2.7451249553777668;-1.754600243050036;0.094882794149762251]
      mask Display: e = 0.06;c1 = [120 150 230]/255;c2 = ([120 150 230]+0)/383;c3 = ([120 150 230]+128)/383;patch([0 1 1 0],[0 0 1 1],c1);patch([0 1 1 1-e 1-e 0+e],[0 0 1 1-e 0+e 0+e],c2);patch([0 0 1 1-e 0+e 0+e],[0 1 1 1-e 1-e 0+e],c3);plot([0 1 1 0 0],[0 0 1 1 0]);disp('Weights');
  "IW{1,1}(10,:)'" : Constant  Value=[-1.0525663617177492;-3.9947523159367657;-3.0103178708532021;-1.5073778774761011;-1.1068577655878524;0.11913174721212702]
      mask Display: e = 0.06;c1 = [120 150 230]/255;c2 = ([120 150 230]+0)/383;c3 = ([120 150 230]+128)/383;patch([0 1 1 0],[0 0 1 1],c1);patch([0 1 1 1-e 1-e 0+e],[0 0 1 1-e 0+e 0+e],c2);patch([0 0 1 1-e 0+e 0+e],[0 1 1 1-e 1-e 0+e],c3);plot([0 1 1 0 0],[0 0 1 1 0]);disp('Weights');
  "IW{1,1}(2,:)'" : Constant  Value=[0.11496507931629137;0.26724308129817653;-1.5649727378899008;-1.4655378549465781;-0.15655593100349188;0.71469015932972868]
      mask Display: e = 0.06;c1 = [120 150 230]/255;c2 = ([120 150 230]+0)/383;c3 = ([120 150 230]+128)/383;patch([0 1 1 0],[0 0 1 1],c1);patch([0 1 1 1-e 1-e 0+e],[0 0 1 1-e 0+e 0+e],c2);patch([0 0 1 1-e 0+e 0+e],[0 1 1 1-e 1-e 0+e],c3);plot([0 1 1 0 0],[0 0 1 1 0]);disp('Weights');
  "IW{1,1}(3,:)'" : Constant  Value=[2.6529527052630262;-0.027691528409082726;-0.86715477642123961;-2.5421217752328458;-3.0166764998421436;0.51956563687730883]
      mask Display: e = 0.06;c1 = [120 150 230]/255;c2 = ([120 150 230]+0)/383;c3 = ([120 150 230]+128)/383;patch([0 1 1 0],[0 0 1 1],c1);patch([0 1 1 1-e 1-e 0+e],[0 0 1 1-e 0+e 0+e],c2);patch([0 0 1 1-e 0+e 0+e],[0 1 1 1-e 1-e 0+e],c3);plot([0 1 1 0 0],[0 0 1 1 0]);disp('Weights');
  "IW{1,1}(4,:)'" : Constant  Value=[1.2651005503765305;1.2422283841670185;1.6659460998232554;0.41969389390695511;2.0509820578160936;1.0180693985491849]
      mask Display: e = 0.06;c1 = [120 150 230]/255;c2 = ([120 150 230]+0)/383;c3 = ([120 150 230]+128)/383;patch([0 1 1 0],[0 0 1 1],c1);patch([0 1 1 1-e 1-e 0+e],[0 0 1 1-e 0+e 0+e],c2);patch([0 0 1 1-e 0+e 0+e],[0 1 1 1-e 1-e 0+e],c3);plot([0 1 1 0 0],[0 0 1 1 0]);disp('Weights');
  "IW{1,1}(5,:)'" : Constant  Value=[-2.7022492940972547;-2.4650425340541062;-1.5485773331809352;-0.71749340971497488;-2.5165455822331912;-0.64233552091618484]
      mask Display: e = 0.06;c1 = [120 150 230]/255;c2 = ([120 150 230]+0)/383;c3 = ([120 150 230]+128)/383;patch([0 1 1 0],[0 0 1 1],c1);patch([0 1 1 1-e 1-e 0+e],[0 0 1 1-e 0+e 0+e],c2);patch([0 0 1 1-e 0+e 0+e],[0 1 1 1-e 1-e 0+e],c3);plot([0 1 1 0 0],[0 0 1 1 0]);disp('Weights');
  "IW{1,1}(6,:)'" : Constant  Value=[-1.636665590828756;-3.4402627061442845;-1.8835695129904932;-1.1572234600596241;-0.87104932773819466;-0.25974609768943696]
      mask Display: e = 0.06;c1 = [120 150 230]/255;c2 = ([120 150 230]+0)/383;c3 = ([120 150 230]+128)/383;patch([0 1 1 0],[0 0 1 1],c1);patch([0 1 1 1-e 1-e 0+e],[0 0 1 1-e 0+e 0+e],c2);patch([0 0 1 1-e 0+e 0+e],[0 1 1 1-e 1-e 0+e],c3);plot([0 1 1 0 0],[0 0 1 1 0]);disp('Weights');
  "IW{1,1}(7,:)'" : Constant  Value=[1.4247404613421883;-0.059934774950113165;-0.68053386512953173;1.4420879465474241;-0.19434467861052421;-0.46806171704165511]
      mask Display: e = 0.06;c1 = [120 150 230]/255;c2 = ([120 150 230]+0)/383;c3 = ([120 150 230]+128)/383;patch([0 1 1 0],[0 0 1 1],c1);patch([0 1 1 1-e 1-e 0+e],[0 0 1 1-e 0+e 0+e],c2);patch([0 0 1 1-e 0+e 0+e],[0 1 1 1-e 1-e 0+e],c3);plot([0 1 1 0 0],[0 0 1 1 0]);disp('Weights');
  "IW{1,1}(8,:)'" : Constant  Value=[1.4549643021986722;-0.16502571404081873;-0.71304431341891639;0.47369961219623241;-1.8599426960293168;1.3816476738965919]
      mask Display: e = 0.06;c1 = [120 150 230]/255;c2 = ([120 150 230]+0)/383;c3 = ([120 150 230]+128)/383;patch([0 1 1 0],[0 0 1 1],c1);patch([0 1 1 1-e 1-e 0+e],[0 0 1 1-e 0+e 0+e],c2);patch([0 0 1 1-e 0+e 0+e],[0 1 1 1-e 1-e 0+e],c3);plot([0 1 1 0 0],[0 0 1 1 0]);disp('Weights');
  "IW{1,1}(9,:)'" : Constant  Value=[-0.48539944278374714;0.020675498189077286;-0.054864128927988642;-0.42269785304866336;1.3501687394567616;1.3700924138975747]
      mask Display: e = 0.06;c1 = [120 150 230]/255;c2 = ([120 150 230]+0)/383;c3 = ([120 150 230]+128)/383;patch([0 1 1 0],[0 0 1 1],c1);patch([0 1 1 1-e 1-e 0+e],[0 0 1 1-e 0+e 0+e],c2);patch([0 0 1 1-e 0+e 0+e],[0 1 1 1-e 1-e 0+e],c3);plot([0 1 1 0 0],[0 0 1 1 0]);disp('Weights');
  Mux : Mux  Inputs=10
      mask Display: e = 0.06;c1 = [120 150 230]/255;c2 = ([120 150 230]+0)/383;c3 = ([120 150 230]+128)/383;patch([0 1 1 0],[0 0 1 1],c1);patch([0 1 1 1-e 1-e 0+e],[0 0 1 1-e 0+e 0+e],c2);patch([0 0 1 1-e 0+e 0+e],[0 1 1 1-e 1-e 0+e],c3);plot([0 1 1 0 0],[0 0 1 1 0]);disp('Mux');
  dotprod{1..10} (10 alike) : neural/Weight Functions/dotprod
  "iz{1,1}" : Outport
      mask Display: e = 0.06;c1 = [120 230 180]/255;c2 = ([120 230 180]+0)/(256+128);c3 = ([120 230 180]+128)/(256+128);patch([0 1 1 0],[0 0 1 1],c1);patch([0 1 1 1-e 1-e 0+e],[0 0 1 1-e 0+e 0+e],c2);patch([0 0 1 1-e 0+e 0+e],[0 1 1 1-e 1-e 0+e],c3);plot([0 1 1 0 0],[0 0 1 1 0]);
  wires:
  "IW{1,1}(1,:)'"/1 -> dotprod1/1
  "pd{1,1}"/1 -> dotprod1/2, dotprod2/2, dotprod3/2, dotprod4/2, dotprod5/2, dotprod6/2, dotprod7/2, dotprod8/2, dotprod9/2, dotprod10/2
  dotprod1/1 -> Mux/1
  "IW{1,1}(2,:)'"/1 -> dotprod2/1
  dotprod2/1 -> Mux/2
  "IW{1,1}(3,:)'"/1 -> dotprod3/1
  dotprod3/1 -> Mux/3
  "IW{1,1}(4,:)'"/1 -> dotprod4/1
  dotprod4/1 -> Mux/4
  "IW{1,1}(5,:)'"/1 -> dotprod5/1
  dotprod5/1 -> Mux/5
  "IW{1,1}(6,:)'"/1 -> dotprod6/1
  dotprod6/1 -> Mux/6
  "IW{1,1}(7,:)'"/1 -> dotprod7/1
  dotprod7/1 -> Mux/7
  "IW{1,1}(8,:)'"/1 -> dotprod8/1
  dotprod8/1 -> Mux/8
  "IW{1,1}(9,:)'"/1 -> dotprod9/1
  dotprod9/1 -> Mux/9
  "IW{1,1}(10,:)'"/1 -> dotprod10/1
  dotprod10/1 -> Mux/10
  Mux/1 -> "iz{1,1}"/1

== system AvonGasTurbineFAult/comp performance/Layer 2/Delays 1 ==
  "p{2}" : Inport  PortDimensions=10
      mask Display: e = 0.06;c1 = [120 230 180]/255;c2 = ([120 230 180]+0)/(256+128);c3 = ([120 230 180]+128)/(256+128);patch([0 1 1 0],[0 0 1 1],c1);patch([0 1 1 1-e 1-e 0+e],[0 0 1 1-e 0+e 0+e],c2);patch([0 0 1 1-e 0+e 0+e],[0 1 1 1-e 1-e 0+e],c3);plot([0 1 1 0 0],[0 0 1 1 0]);
  mux : Mux  Inputs=1
      mask Display: e = 0.06;c1 = [120 150 230]/255;c2 = ([120 150 230]+0)/383;c3 = ([120 150 230]+128)/383;patch([0 1 1 0],[0 0 1 1],c1);patch([0 1 1 1-e 1-e 0+e],[0 0 1 1-e 0+e 0+e],c2);patch([0 0 1 1-e 0+e 0+e],[0 1 1 1-e 1-e 0+e],c3);plot([0 1 1 0 0],[0 0 1 1 0]);disp('Mux')
  "pd{2,1}" : Outport
      mask Display: e = 0.06;c1 = [120 230 180]/255;c2 = ([120 230 180]+0)/(256+128);c3 = ([120 230 180]+128)/(256+128);patch([0 1 1 0],[0 0 1 1],c1);patch([0 1 1 1-e 1-e 0+e],[0 0 1 1-e 0+e 0+e],c2);patch([0 0 1 1-e 0+e 0+e],[0 1 1 1-e 1-e 0+e],c3);plot([0 1 1 0 0],[0 0 1 1 0]);
  wires:
  "p{2}"/1 -> mux/1
  mux/1 -> "pd{2,1}"/1

== system AvonGasTurbineFAult/comp performance/Layer 2/LW{2,1} ==
  "ad{2,1}" : Inport  PortDimensions=10
      mask Display: e = 0.06;c1 = [120 230 180]/255;c2 = ([120 230 180]+0)/(256+128);c3 = ([120 230 180]+128)/(256+128);patch([0 1 1 0],[0 0 1 1],c1);patch([0 1 1 1-e 1-e 0+e],[0 0 1 1-e 0+e 0+e],c2);patch([0 0 1 1-e 0+e 0+e],[0 1 1 1-e 1-e 0+e],c3);plot([0 1 1 0 0],[0 0 1 1 0]);
  "IW{2,1}(1,:)'" : Constant  Value=[4.4431695764236006;0.35588224738583341;-4.4391058278770918;0.51998224828591522;-0.87087923132958356;2.5069740300413077;0.45699494303394589;-1.9702170905255949;1.6365102022594566;1.0757230457059122]
      mask Display: e = 0.06;c1 = [120 150 230]/255;c2 = ([120 150 230]+0)/383;c3 = ([120 150 230]+128)/383;patch([0 1 1 0],[0 0 1 1],c1);patch([0 1 1 1-e 1-e 0+e],[0 0 1 1-e 0+e 0+e],c2);patch([0 0 1 1-e 0+e 0+e],[0 1 1 1-e 1-e 0+e],c3);plot([0 1 1 0 0],[0 0 1 1 0]);disp('weights');
  "IW{2,1}(2,:)'" : Constant  Value=[-4.20197557037622;0.37168986646841223;-0.82168117276682862;1.4011177395692749;-0.86413368466618945;5.9723736459165231;1.0079702028586519;0.37479064156139574;1.8543987569738158;3.0102939655396663]
      mask Display: e = 0.06;c1 = [120 150 230]/255;c2 = ([120 150 230]+0)/383;c3 = ([120 150 230]+128)/383;patch([0 1 1 0],[0 0 1 1],c1);patch([0 1 1 1-e 1-e 0+e],[0 0 1 1-e 0+e 0+e],c2);patch([0 0 1 1-e 0+e 0+e],[0 1 1 1-e 1-e 0+e],c3);plot([0 1 1 0 0],[0 0 1 1 0]);disp('weights');
  "IW{2,1}(3,:)'" : Constant  Value=[-3.0935796983956161;0.15596024012571752;1.5886948976133448;-0.40452876958428741;1.1649129261609081;3.0362030303885081;0.035719228902631517;0.53487772784294207;-0.5527710288195874;-4.3630446314384921]
      mask Display: e = 0.06;c1 = [120 150 230]/255;c2 = ([120 150 230]+0)/383;c3 = ([120 150 230]+128)/383;patch([0 1 1 0],[0 0 1 1],c1);patch([0 1 1 1-e 1-e 0+e],[0 0 1 1-e 0+e 0+e],c2);patch([0 0 1 1-e 0+e 0+e],[0 1 1 1-e 1-e 0+e],c3);plot([0 1 1 0 0],[0 0 1 1 0]);disp('weights');
  "IW{2,1}(4,:)'" : Constant  Value=[0.017571754787948542;0.40843882036648438;0.39733331510868808;-2.0076896675518405;2.9503549974222119;-5.576119385144513;0.13813434766481739;0.12357378061532175;-0.58539699991680127;-1.6525295777788587]
      mask Display: e = 0.06;c1 = [120 150 230]/255;c2 = ([120 150 230]+0)/383;c3 = ([120 150 230]+128)/383;patch([0 1 1 0],[0 0 1 1],c1);patch([0 1 1 1-e 1-e 0+e],[0 0 1 1-e 0+e 0+e],c2);patch([0 0 1 1-e 0+e 0+e],[0 1 1 1-e 1-e 0+e],c3);plot([0 1 1 0 0],[0 0 1 1 0]);disp('weights');
  "IW{2,1}(5,:)'" : Constant  Value=[2.0121820205661765;-0.94247097353891307;1.485114318468479;1.4313381770709912;-2.9248522976429263;-4.4507876166853375;0.41565702298567675;0.058415223148058637;-2.7847231810154294;-0.21968219503925385]
      mask Display: e = 0.06;c1 = [120 150 230]/255;c2 = ([120 150 230]+0)/383;c3 = ([120 150 230]+128)/383;patch([0 1 1 0],[0 0 1 1],c1);patch([0 1 1 1-e 1-e 0+e],[0 0 1 1-e 0+e 0+e],c2);patch([0 0 1 1-e 0+e 0+e],[0 1 1 1-e 1-e 0+e],c3);plot([0 1 1 0 0],[0 0 1 1 0]);disp('weights');
  Mux : Mux  Inputs=5
      mask Display: e = 0.06;c1 = [120 150 230]/255;c2 = ([120 150 230]+0)/383;c3 = ([120 150 230]+128)/383;patch([0 1 1 0],[0 0 1 1],c1);patch([0 1 1 1-e 1-e 0+e],[0 0 1 1-e 0+e 0+e],c2);patch([0 0 1 1-e 0+e 0+e],[0 1 1 1-e 1-e 0+e],c3);plot([0 1 1 0 0],[0 0 1 1 0]);disp('Mux');
  dotprod{1..5} (5 alike) : neural/Weight Functions/dotprod
  "lz{2,1}" : Outport
      mask Display: e = 0.06;c1 = [120 230 180]/255;c2 = ([120 230 180]+0)/(256+128);c3 = ([120 230 180]+128)/(256+128);patch([0 1 1 0],[0 0 1 1],c1);patch([0 1 1 1-e 1-e 0+e],[0 0 1 1-e 0+e 0+e],c2);patch([0 0 1 1-e 0+e 0+e],[0 1 1 1-e 1-e 0+e],c3);plot([0 1 1 0 0],[0 0 1 1 0]);
  wires:
  "IW{2,1}(1,:)'"/1 -> dotprod1/1
  "ad{2,1}"/1 -> dotprod1/2, dotprod2/2, dotprod3/2, dotprod4/2, dotprod5/2
  dotprod1/1 -> Mux/1
  "IW{2,1}(2,:)'"/1 -> dotprod2/1
  dotprod2/1 -> Mux/2
  "IW{2,1}(3,:)'"/1 -> dotprod3/1
  dotprod3/1 -> Mux/3
  "IW{2,1}(4,:)'"/1 -> dotprod4/1
  dotprod4/1 -> Mux/4
  "IW{2,1}(5,:)'"/1 -> dotprod5/1
  dotprod5/1 -> Mux/5
  Mux/1 -> "lz{2,1}"/1
